simulink model "bmsTestPlatform"  (R2025b)
settings: configuration reference "cfgHarness" (kept outside this file)
PreLoadFcn:
  | if isempty(matlab.project.rootProject)
  |     % Opened outside the project (e.g. by RT-LAB): open it, then return to this folder
  |     d = pwd;
  |     try, openProject(fullfile(d, "..")); catch e, warning(e.message); end
  |     cd(d);
  | end
InitFcn:
  | plant_params
  | sensor_params
  | load_params
undefined symbols (not defined in the file): ADV_tStale, ARB_socTol, batMod, battery_builder_rtmsupport, BMS_state, BMS_stubOut, CAN_Ts, DiscIntNeverNeededParam, f, gcbh, HW_nvm, HW_powerPress, HW_resetPress, HW_rtcStart, LOAD_cycleA, LOAD_cycleAext, LOAD_iConst, LOAD_iPulse, LOAD_profile, LOAD_pulseDuty, LOAD_pulsePeriod, LOAD_scale, PLANT_switchFault, PLANT_tAmbient, PLANT_tContactor, PLANT_Ts, sens, SENS_faultChannel, SENS_faultDuration, SENS_faultRamp, SENS_faultStart, SENS_faultType, SENS_faultValue, SOC0, T0
libraries: bat_13S7P_detailed_lib x7, fl_lib x5, nesl_utility x4, simulink x3, instrumentlib x2
(part 2 of 2)

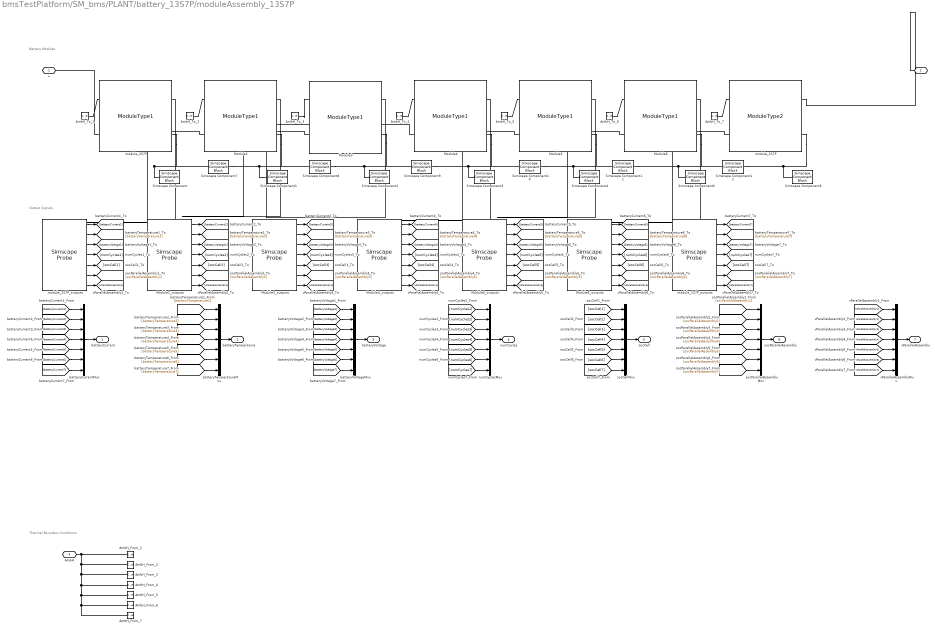
== system bmsTestPlatform/SM_bms/PLANT/battery_13S7P/moduleAssembly_13S7P ==
  note: Thermal Boundary Conditions
  note: Output Signals
  note: Battery Modules
  AmbH_From_1 : ConnectionLabel  Label=ambH_1
  AmbH_From_2 : ConnectionLabel  Label=ambH_2
  AmbH_From_3 : ConnectionLabel  Label=ambH_3
  AmbH_From_4 : ConnectionLabel  Label=ambH_4
  AmbH_From_5 : ConnectionLabel  Label=ambH_5
  AmbH_From_6 : ConnectionLabel  Label=ambH_6
  AmbH_From_7 : ConnectionLabel  Label=ambH_7
  AmbH_To_1 : ConnectionLabel  Label=ambH_1
  AmbH_To_2 : ConnectionLabel  Label=ambH_2
  AmbH_To_3 : ConnectionLabel  Label=ambH_3
  AmbH_To_4 : ConnectionLabel  Label=ambH_4
  AmbH_To_5 : ConnectionLabel  Label=ambH_5
  AmbH_To_6 : ConnectionLabel  Label=ambH_6
  AmbH_To_7 : ConnectionLabel  Label=ambH_7
  Module2 : bat_13S7P_detailed_lib/Modules/ModuleType1  BatteryCapacityCell=batMod(2).BatteryCapacityCell A*hr  ExtrapolationMethodCell=simscape.enum.extrapolation.nearest  SOCBreakpointsCell=batMod(2).SOCBreakpointsCell  TemperatureBreakpointsCell=batMod(2).TemperatureBreakpointsCell K  OpenCircuitVoltageThermalCell=batMod(2).OpenCircuitVoltageThermalCell V  VoltageRangeCell=batMod(2).VoltageRangeCell V  ResistanceSOCBreakpointsCell=batMod(2).ResistanceSOCBreakpointsCell  ResistanceTemperatureBreakpointsCell=batMod(2).ResistanceTemperatureBreakpointsCell K  R0ThermalCell=batMod(2).R0ThermalCell Ohm  R1ThermalCell=batMod(2).R1ThermalCell Ohm  Tau1ThermalCell=batMod(2).Tau1ThermalCell s  BatteryThermalMassCell=batMod(2).BatteryThermalMassCell J/K  AmbientResistance=batMod(2).AmbientResistance K/W  P=7  S=2  socCell_specify=on  socCell_priority=High  socCell=SOC0*ones(14,1)  socCell_nominal_specify=off  socCell_nominal_value=1  socCell_nominal_unit=1  batteryVoltage_specify=off  batteryVoltage_priority=None  batteryVoltage=repmat(0, 14, 1) V  batteryVoltage_nominal_specify=off  batteryVoltage_nominal_value=1  batteryVoltage_nominal_unit=V  batteryCurrent_specify=off  batteryCurrent_priority=None  batteryCurrent=repmat(0, 14, 1) A  batteryCurrent_nominal_specify=off  batteryCurrent_nominal_value=1  batteryCurrent_nominal_unit=A  numCycles_specify=off  numCycles_priority=High  numCycles=repmat(0, 14, 1)  numCycles_nominal_specify=off  numCycles_nominal_value=1  numCycles_nominal_unit=1  batteryTemperature_specify=on  batteryTemperature_priority=High  batteryTemperature=T0*ones(14,1) K  batteryTemperature_nominal_specify=off  batteryTemperature_nominal_value=1  batteryTemperature_nominal_unit=K  vParallelAssembly_specify=off  vParallelAssembly_priority=None  vParallelAssembly=repmat(0, 2, 1) V  vParallelAssembly_nominal_specify=off  vParallelAssembly_nominal_value=1  vParallelAssembly_nominal_unit=V  socParallelAssembly_specify=off  socParallelAssembly_priority=None  socParallelAssembly=repmat(1, 2, 1)  socParallelAssembly_nominal_specify=off  socParallelAssembly_nominal_value=1  socParallelAssembly_nominal_unit=1
      settings: InternalSimscapePortConfiguration="{\"Bottom\":[{\"id\":\"n\",\"label\":\"-\",\"type\":\"foundation.electrical.electrical\"},{\"id\":\"BottomExtClnt\",\"label\":\"CPB\",\"type\":\"foundation.thermal.thermal\"}],\"Left\":[{\"id\":\"AmbH\",\"label\":\"AmbH\",\"type\":\"foundation.thermal.thermal\"}],\"Right\":[],\"Top\":[{\"id\":\"p\",\"label\":\"+\",\"type\":\"foundation.electrical.electrical\"}]}"
  Module2_outputs : SimscapeProbe  BoundBlock=68  Variables="{\"batteryCurrent\":{\"Probing\":\"ON\"},\"batteryTemperature\":{\"Probing\":\"ON\"},\"batteryVoltage\":{\"Probing\":\"ON\"},\"numCycles\":{\"Probing\":\"ON\"},\"socCell\":{\"Probing\":\"ON\"},\"socParallelAssembly\":{\"Probing\":\"ON\"},\"vParallelAssembly\":{\"Probing\":\"ON\"}}"
  Module3 : bat_13S7P_detailed_lib/Modules/ModuleType1  BatteryCapacityCell=batMod(3).BatteryCapacityCell A*hr  ExtrapolationMethodCell=simscape.enum.extrapolation.nearest  SOCBreakpointsCell=batMod(3).SOCBreakpointsCell  TemperatureBreakpointsCell=batMod(3).TemperatureBreakpointsCell K  OpenCircuitVoltageThermalCell=batMod(3).OpenCircuitVoltageThermalCell V  VoltageRangeCell=batMod(3).VoltageRangeCell V  ResistanceSOCBreakpointsCell=batMod(3).ResistanceSOCBreakpointsCell  ResistanceTemperatureBreakpointsCell=batMod(3).ResistanceTemperatureBreakpointsCell K  R0ThermalCell=batMod(3).R0ThermalCell Ohm  R1ThermalCell=batMod(3).R1ThermalCell Ohm  Tau1ThermalCell=batMod(3).Tau1ThermalCell s  BatteryThermalMassCell=batMod(3).BatteryThermalMassCell J/K  AmbientResistance=batMod(3).AmbientResistance K/W  P=7  S=2  socCell_specify=on  socCell_priority=High  socCell=SOC0*ones(14,1)  socCell_nominal_specify=off  socCell_nominal_value=1  socCell_nominal_unit=1  batteryVoltage_specify=off  batteryVoltage_priority=None  batteryVoltage=repmat(0, 14, 1) V  batteryVoltage_nominal_specify=off  batteryVoltage_nominal_value=1  batteryVoltage_nominal_unit=V  batteryCurrent_specify=off  batteryCurrent_priority=None  batteryCurrent=repmat(0, 14, 1) A  batteryCurrent_nominal_specify=off  batteryCurrent_nominal_value=1  batteryCurrent_nominal_unit=A  numCycles_specify=off  numCycles_priority=High  numCycles=repmat(0, 14, 1)  numCycles_nominal_specify=off  numCycles_nominal_value=1  numCycles_nominal_unit=1  batteryTemperature_specify=on  batteryTemperature_priority=High  batteryTemperature=T0*ones(14,1) K  batteryTemperature_nominal_specify=off  batteryTemperature_nominal_value=1  batteryTemperature_nominal_unit=K  vParallelAssembly_specify=off  vParallelAssembly_priority=None  vParallelAssembly=repmat(0, 2, 1) V  vParallelAssembly_nominal_specify=off  vParallelAssembly_nominal_value=1  vParallelAssembly_nominal_unit=V  socParallelAssembly_specify=off  socParallelAssembly_priority=None  socParallelAssembly=repmat(1, 2, 1)  socParallelAssembly_nominal_specify=off  socParallelAssembly_nominal_value=1  socParallelAssembly_nominal_unit=1
      settings: InternalSimscapePortConfiguration="{\"Bottom\":[{\"id\":\"n\",\"label\":\"-\",\"type\":\"foundation.electrical.electrical\"},{\"id\":\"BottomExtClnt\",\"label\":\"CPB\",\"type\":\"foundation.thermal.thermal\"}],\"Left\":[{\"id\":\"AmbH\",\"label\":\"AmbH\",\"type\":\"foundation.thermal.thermal\"}],\"Right\":[],\"Top\":[{\"id\":\"p\",\"label\":\"+\",\"type\":\"foundation.electrical.electrical\"}]}"
  Module3_outputs : SimscapeProbe  BoundBlock=70  Variables="{\"batteryCurrent\":{\"Probing\":\"ON\"},\"batteryTemperature\":{\"Probing\":\"ON\"},\"batteryVoltage\":{\"Probing\":\"ON\"},\"numCycles\":{\"Probing\":\"ON\"},\"socCell\":{\"Probing\":\"ON\"},\"socParallelAssembly\":{\"Probing\":\"ON\"},\"vParallelAssembly\":{\"Probing\":\"ON\"}}"
  Module4 : bat_13S7P_detailed_lib/Modules/ModuleType1  BatteryCapacityCell=batMod(4).BatteryCapacityCell A*hr  ExtrapolationMethodCell=simscape.enum.extrapolation.nearest  SOCBreakpointsCell=batMod(4).SOCBreakpointsCell  TemperatureBreakpointsCell=batMod(4).TemperatureBreakpointsCell K  OpenCircuitVoltageThermalCell=batMod(4).OpenCircuitVoltageThermalCell V  VoltageRangeCell=batMod(4).VoltageRangeCell V  ResistanceSOCBreakpointsCell=batMod(4).ResistanceSOCBreakpointsCell  ResistanceTemperatureBreakpointsCell=batMod(4).ResistanceTemperatureBreakpointsCell K  R0ThermalCell=batMod(4).R0ThermalCell Ohm  R1ThermalCell=batMod(4).R1ThermalCell Ohm  Tau1ThermalCell=batMod(4).Tau1ThermalCell s  BatteryThermalMassCell=batMod(4).BatteryThermalMassCell J/K  AmbientResistance=batMod(4).AmbientResistance K/W  P=7  S=2  socCell_specify=on  socCell_priority=High  socCell=SOC0*ones(14,1)  socCell_nominal_specify=off  socCell_nominal_value=1  socCell_nominal_unit=1  batteryVoltage_specify=off  batteryVoltage_priority=None  batteryVoltage=repmat(0, 14, 1) V  batteryVoltage_nominal_specify=off  batteryVoltage_nominal_value=1  batteryVoltage_nominal_unit=V  batteryCurrent_specify=off  batteryCurrent_priority=None  batteryCurrent=repmat(0, 14, 1) A  batteryCurrent_nominal_specify=off  batteryCurrent_nominal_value=1  batteryCurrent_nominal_unit=A  numCycles_specify=off  numCycles_priority=High  numCycles=repmat(0, 14, 1)  numCycles_nominal_specify=off  numCycles_nominal_value=1  numCycles_nominal_unit=1  batteryTemperature_specify=on  batteryTemperature_priority=High  batteryTemperature=T0*ones(14,1) K  batteryTemperature_nominal_specify=off  batteryTemperature_nominal_value=1  batteryTemperature_nominal_unit=K  vParallelAssembly_specify=off  vParallelAssembly_priority=None  vParallelAssembly=repmat(0, 2, 1) V  vParallelAssembly_nominal_specify=off  vParallelAssembly_nominal_value=1  vParallelAssembly_nominal_unit=V  socParallelAssembly_specify=off  socParallelAssembly_priority=None  socParallelAssembly=repmat(1, 2, 1)  socParallelAssembly_nominal_specify=off  socParallelAssembly_nominal_value=1  socParallelAssembly_nominal_unit=1
      settings: InternalSimscapePortConfiguration="{\"Bottom\":[{\"id\":\"n\",\"label\":\"-\",\"type\":\"foundation.electrical.electrical\"},{\"id\":\"BottomExtClnt\",\"label\":\"CPB\",\"type\":\"foundation.thermal.thermal\"}],\"Left\":[{\"id\":\"AmbH\",\"label\":\"AmbH\",\"type\":\"foundation.thermal.thermal\"}],\"Right\":[],\"Top\":[{\"id\":\"p\",\"label\":\"+\",\"type\":\"foundation.electrical.electrical\"}]}"
  Module4_outputs : SimscapeProbe  BoundBlock=72  Variables="{\"batteryCurrent\":{\"Probing\":\"ON\"},\"batteryTemperature\":{\"Probing\":\"ON\"},\"batteryVoltage\":{\"Probing\":\"ON\"},\"numCycles\":{\"Probing\":\"ON\"},\"socCell\":{\"Probing\":\"ON\"},\"socParallelAssembly\":{\"Probing\":\"ON\"},\"vParallelAssembly\":{\"Probing\":\"ON\"}}"
  Module5 : bat_13S7P_detailed_lib/Modules/ModuleType1  BatteryCapacityCell=batMod(5).BatteryCapacityCell A*hr  ExtrapolationMethodCell=simscape.enum.extrapolation.nearest  SOCBreakpointsCell=batMod(5).SOCBreakpointsCell  TemperatureBreakpointsCell=batMod(5).TemperatureBreakpointsCell K  OpenCircuitVoltageThermalCell=batMod(5).OpenCircuitVoltageThermalCell V  VoltageRangeCell=batMod(5).VoltageRangeCell V  ResistanceSOCBreakpointsCell=batMod(5).ResistanceSOCBreakpointsCell  ResistanceTemperatureBreakpointsCell=batMod(5).ResistanceTemperatureBreakpointsCell K  R0ThermalCell=batMod(5).R0ThermalCell Ohm  R1ThermalCell=batMod(5).R1ThermalCell Ohm  Tau1ThermalCell=batMod(5).Tau1ThermalCell s  BatteryThermalMassCell=batMod(5).BatteryThermalMassCell J/K  AmbientResistance=batMod(5).AmbientResistance K/W  P=7  S=2  socCell_specify=on  socCell_priority=High  socCell=SOC0*ones(14,1)  socCell_nominal_specify=off  socCell_nominal_value=1  socCell_nominal_unit=1  batteryVoltage_specify=off  batteryVoltage_priority=None  batteryVoltage=repmat(0, 14, 1) V  batteryVoltage_nominal_specify=off  batteryVoltage_nominal_value=1  batteryVoltage_nominal_unit=V  batteryCurrent_specify=off  batteryCurrent_priority=None  batteryCurrent=repmat(0, 14, 1) A  batteryCurrent_nominal_specify=off  batteryCurrent_nominal_value=1  batteryCurrent_nominal_unit=A  numCycles_specify=off  numCycles_priority=High  numCycles=repmat(0, 14, 1)  numCycles_nominal_specify=off  numCycles_nominal_value=1  numCycles_nominal_unit=1  batteryTemperature_specify=on  batteryTemperature_priority=High  batteryTemperature=T0*ones(14,1) K  batteryTemperature_nominal_specify=off  batteryTemperature_nominal_value=1  batteryTemperature_nominal_unit=K  vParallelAssembly_specify=off  vParallelAssembly_priority=None  vParallelAssembly=repmat(0, 2, 1) V  vParallelAssembly_nominal_specify=off  vParallelAssembly_nominal_value=1  vParallelAssembly_nominal_unit=V  socParallelAssembly_specify=off  socParallelAssembly_priority=None  socParallelAssembly=repmat(1, 2, 1)  socParallelAssembly_nominal_specify=off  socParallelAssembly_nominal_value=1  socParallelAssembly_nominal_unit=1
      settings: InternalSimscapePortConfiguration="{\"Bottom\":[{\"id\":\"n\",\"label\":\"-\",\"type\":\"foundation.electrical.electrical\"},{\"id\":\"BottomExtClnt\",\"label\":\"CPB\",\"type\":\"foundation.thermal.thermal\"}],\"Left\":[{\"id\":\"AmbH\",\"label\":\"AmbH\",\"type\":\"foundation.thermal.thermal\"}],\"Right\":[],\"Top\":[{\"id\":\"p\",\"label\":\"+\",\"type\":\"foundation.electrical.electrical\"}]}"
  Module5_outputs : SimscapeProbe  BoundBlock=74  Variables="{\"batteryCurrent\":{\"Probing\":\"ON\"},\"batteryTemperature\":{\"Probing\":\"ON\"},\"batteryVoltage\":{\"Probing\":\"ON\"},\"numCycles\":{\"Probing\":\"ON\"},\"socCell\":{\"Probing\":\"ON\"},\"socParallelAssembly\":{\"Probing\":\"ON\"},\"vParallelAssembly\":{\"Probing\":\"ON\"}}"
  Module6 : bat_13S7P_detailed_lib/Modules/ModuleType1  BatteryCapacityCell=batMod(6).BatteryCapacityCell A*hr  ExtrapolationMethodCell=simscape.enum.extrapolation.nearest  SOCBreakpointsCell=batMod(6).SOCBreakpointsCell  TemperatureBreakpointsCell=batMod(6).TemperatureBreakpointsCell K  OpenCircuitVoltageThermalCell=batMod(6).OpenCircuitVoltageThermalCell V  VoltageRangeCell=batMod(6).VoltageRangeCell V  ResistanceSOCBreakpointsCell=batMod(6).ResistanceSOCBreakpointsCell  ResistanceTemperatureBreakpointsCell=batMod(6).ResistanceTemperatureBreakpointsCell K  R0ThermalCell=batMod(6).R0ThermalCell Ohm  R1ThermalCell=batMod(6).R1ThermalCell Ohm  Tau1ThermalCell=batMod(6).Tau1ThermalCell s  BatteryThermalMassCell=batMod(6).BatteryThermalMassCell J/K  AmbientResistance=batMod(6).AmbientResistance K/W  P=7  S=2  socCell_specify=on  socCell_priority=High  socCell=SOC0*ones(14,1)  socCell_nominal_specify=off  socCell_nominal_value=1  socCell_nominal_unit=1  batteryVoltage_specify=off  batteryVoltage_priority=None  batteryVoltage=repmat(0, 14, 1) V  batteryVoltage_nominal_specify=off  batteryVoltage_nominal_value=1  batteryVoltage_nominal_unit=V  batteryCurrent_specify=off  batteryCurrent_priority=None  batteryCurrent=repmat(0, 14, 1) A  batteryCurrent_nominal_specify=off  batteryCurrent_nominal_value=1  batteryCurrent_nominal_unit=A  numCycles_specify=off  numCycles_priority=High  numCycles=repmat(0, 14, 1)  numCycles_nominal_specify=off  numCycles_nominal_value=1  numCycles_nominal_unit=1  batteryTemperature_specify=on  batteryTemperature_priority=High  batteryTemperature=T0*ones(14,1) K  batteryTemperature_nominal_specify=off  batteryTemperature_nominal_value=1  batteryTemperature_nominal_unit=K  vParallelAssembly_specify=off  vParallelAssembly_priority=None  vParallelAssembly=repmat(0, 2, 1) V  vParallelAssembly_nominal_specify=off  vParallelAssembly_nominal_value=1  vParallelAssembly_nominal_unit=V  socParallelAssembly_specify=off  socParallelAssembly_priority=None  socParallelAssembly=repmat(1, 2, 1)  socParallelAssembly_nominal_specify=off  socParallelAssembly_nominal_value=1  socParallelAssembly_nominal_unit=1
      settings: InternalSimscapePortConfiguration="{\"Bottom\":[{\"id\":\"n\",\"label\":\"-\",\"type\":\"foundation.electrical.electrical\"},{\"id\":\"BottomExtClnt\",\"label\":\"CPB\",\"type\":\"foundation.thermal.thermal\"}],\"Left\":[{\"id\":\"AmbH\",\"label\":\"AmbH\",\"type\":\"foundation.thermal.thermal\"}],\"Right\":[],\"Top\":[{\"id\":\"p\",\"label\":\"+\",\"type\":\"foundation.electrical.electrical\"}]}"
  Module6_outputs : SimscapeProbe  BoundBlock=76  Variables="{\"batteryCurrent\":{\"Probing\":\"ON\"},\"batteryTemperature\":{\"Probing\":\"ON\"},\"batteryVoltage\":{\"Probing\":\"ON\"},\"numCycles\":{\"Probing\":\"ON\"},\"socCell\":{\"Probing\":\"ON\"},\"socParallelAssembly\":{\"Probing\":\"ON\"},\"vParallelAssembly\":{\"Probing\":\"ON\"}}"
  Simscape Component{,1..5} (6 alike) : SimscapeComponentBlock  SourceFile=cellPairs_2S7P  ComponentPath=cellPairs_2S7P  ComponentVariants="[\"cellPairs_2S7P\"]"  ComponentVariantNames="[\"cellPairs_2S7P\"]"  ClassName=cellPairs_2S7P  SchemaVersion=1  R=[61.73, 54.15, 61.73, 57.32, 61.72, 58.62, 58.63, 55.64, 58.64, 55.64, 58.63, 61.72, 58.62, 57.32, 54.15, 61.73, 61.73] K/W
      settings: CopyFcn=simscape.sscblock.internal.componentBlockCallback(gcbh,'COPY')  PreCopyFcn=simscape.sscblock.internal.componentBlockCallback(gcbh,'PRECOPY')  PreDeleteFcn=simscape.sscblock.internal.componentBlockCallback(gcbh,'PREDELETE')  InternalSimscapePortConfiguration="{\"Bottom\":[],\"Left\":[{\"id\":\"H\",\"label\":\"H\",\"type\":\"foundation.thermal.thermal\"}],\"Right\":[],\"Top\":[]}"
      mask Type: Cell-to-cell thermal network within one 2S7P slice (14 cells, 17 neighbour pairs).
  Simscape Component{7..11} (5 alike) : SimscapeComponentBlock  SourceFile=axialLink_2S7P  ComponentPath=axialLink_2S7P  ComponentVariants="[\"axialLink_2S7P\"]"  ComponentVariantNames="[\"axialLink_2S7P\"]"  ClassName=axialLink_2S7P  SchemaVersion=1  R=180.4 K/W
      settings: CopyFcn=simscape.sscblock.internal.componentBlockCallback(gcbh,'COPY')  PreCopyFcn=simscape.sscblock.internal.componentBlockCallback(gcbh,'PRECOPY')  PreDeleteFcn=simscape.sscblock.internal.componentBlockCallback(gcbh,'PREDELETE')  InternalSimscapePortConfiguration="{\"Bottom\":[],\"Left\":[{\"id\":\"A\",\"label\":\"A\",\"type\":\"foundation.thermal.thermal\"}],\"Right\":[{\"id\":\"B\",\"label\":\"B\",\"type\":\"foundation.thermal.thermal\"}],\"Top\":[]}"
      mask Type: Slice-to-slice thermal links
  Simscape Component12 : SimscapeComponentBlock  SourceFile=axialLink_2S7P_1S7P  ComponentPath=axialLink_2S7P_1S7P  ComponentVariants="[\"axialLink_2S7P_1S7P\"]"  ComponentVariantNames="[\"axialLink_2S7P_1S7P\"]"  ClassName=axialLink_2S7P_1S7P  SchemaVersion=1  R=180.4 K/W
      settings: CopyFcn=simscape.sscblock.internal.componentBlockCallback(gcbh,'COPY')  PreCopyFcn=simscape.sscblock.internal.componentBlockCallback(gcbh,'PRECOPY')  PreDeleteFcn=simscape.sscblock.internal.componentBlockCallback(gcbh,'PREDELETE')  InternalSimscapePortConfiguration="{\"Bottom\":[],\"Left\":[{\"id\":\"A\",\"label\":\"A\",\"type\":\"foundation.thermal.thermal\"}],\"Right\":[{\"id\":\"B\",\"label\":\"B\",\"type\":\"foundation.thermal.thermal\"}],\"Top\":[]}"
      mask Type: Slice-to-slice thermal links
  Simscape Component6 : SimscapeComponentBlock  SourceFile=cellPairs_1S7P  ComponentPath=cellPairs_1S7P  ComponentVariants="[\"cellPairs_1S7P\"]"  ComponentVariantNames="[\"cellPairs_1S7P\"]"  ClassName=cellPairs_1S7P  SchemaVersion=1  R=[61.73, 54.15, 61.73, 57.32, 61.72, 58.62, 58.63, 55.64] K/W
      settings: CopyFcn=simscape.sscblock.internal.componentBlockCallback(gcbh,'COPY')  PreCopyFcn=simscape.sscblock.internal.componentBlockCallback(gcbh,'PRECOPY')  PreDeleteFcn=simscape.sscblock.internal.componentBlockCallback(gcbh,'PREDELETE')  InternalSimscapePortConfiguration="{\"Bottom\":[],\"Left\":[{\"id\":\"H\",\"label\":\"H\",\"type\":\"foundation.thermal.thermal\"}],\"Right\":[],\"Top\":[]}"
      mask Type: Cell-to-cell thermal network within one 1S7P slice (7 cells, 8 neighbour pairs).
  batteryCurrentMux : Mux  Inputs=7
  batteryTemperatureMux : Mux  Inputs=7
  batteryVoltageMux : Mux  Inputs=7
  module_1S7P : bat_13S7P_detailed_lib/Modules/ModuleType2  BatteryCapacityCell=batMod(7).BatteryCapacityCell A*hr  ExtrapolationMethodCell=simscape.enum.extrapolation.nearest  SOCBreakpointsCell=batMod(7).SOCBreakpointsCell  TemperatureBreakpointsCell=batMod(7).TemperatureBreakpointsCell K  OpenCircuitVoltageThermalCell=batMod(7).OpenCircuitVoltageThermalCell V  VoltageRangeCell=batMod(7).VoltageRangeCell V  ResistanceSOCBreakpointsCell=batMod(7).ResistanceSOCBreakpointsCell  ResistanceTemperatureBreakpointsCell=batMod(7).ResistanceTemperatureBreakpointsCell K  R0ThermalCell=batMod(7).R0ThermalCell Ohm  R1ThermalCell=batMod(7).R1ThermalCell Ohm  Tau1ThermalCell=batMod(7).Tau1ThermalCell s  BatteryThermalMassCell=batMod(7).BatteryThermalMassCell J/K  AmbientResistance=batMod(7).AmbientResistance K/W  P=7  S=1  socCell_specify=on  socCell_priority=High  socCell=SOC0*ones(7,1)  socCell_nominal_specify=off  socCell_nominal_value=1  socCell_nominal_unit=1  batteryVoltage_specify=off  batteryVoltage_priority=None  batteryVoltage=repmat(0, 7, 1) V  batteryVoltage_nominal_specify=off  batteryVoltage_nominal_value=1  batteryVoltage_nominal_unit=V  batteryCurrent_specify=off  batteryCurrent_priority=None  batteryCurrent=repmat(0, 7, 1) A  batteryCurrent_nominal_specify=off  batteryCurrent_nominal_value=1  batteryCurrent_nominal_unit=A  numCycles_specify=off  numCycles_priority=High  numCycles=repmat(0, 7, 1)  numCycles_nominal_specify=off  numCycles_nominal_value=1  numCycles_nominal_unit=1  batteryTemperature_specify=on  batteryTemperature_priority=High  batteryTemperature=T0*ones(7,1) K  batteryTemperature_nominal_specify=off  batteryTemperature_nominal_value=1  batteryTemperature_nominal_unit=K  vParallelAssembly_specify=off  vParallelAssembly_priority=None  vParallelAssembly=0 V  vParallelAssembly_nominal_specify=off  vParallelAssembly_nominal_value=1  vParallelAssembly_nominal_unit=V  socParallelAssembly_specify=off  socParallelAssembly_priority=None  socParallelAssembly=1  socParallelAssembly_nominal_specify=off  socParallelAssembly_nominal_value=1  socParallelAssembly_nominal_unit=1
      settings: InternalSimscapePortConfiguration="{\"Bottom\":[{\"id\":\"n\",\"label\":\"-\",\"type\":\"foundation.electrical.electrical\"},{\"id\":\"BottomExtClnt\",\"label\":\"CPB\",\"type\":\"foundation.thermal.thermal\"}],\"Left\":[{\"id\":\"AmbH\",\"label\":\"AmbH\",\"type\":\"foundation.thermal.thermal\"}],\"Right\":[],\"Top\":[{\"id\":\"p\",\"label\":\"+\",\"type\":\"foundation.electrical.electrical\"}]}"
  module_1S7P_outputs : SimscapeProbe  BoundBlock=123  Variables="{\"batteryCurrent\":{\"Probing\":\"ON\"},\"batteryTemperature\":{\"Probing\":\"ON\"},\"batteryVoltage\":{\"Probing\":\"ON\"},\"numCycles\":{\"Probing\":\"ON\"},\"socCell\":{\"Probing\":\"ON\"},\"socParallelAssembly\":{\"Probing\":\"ON\"},\"vParallelAssembly\":{\"Probing\":\"ON\"}}"
  module_2S7P : bat_13S7P_detailed_lib/Modules/ModuleType1  BatteryCapacityCell=batMod(1).BatteryCapacityCell A*hr  ExtrapolationMethodCell=simscape.enum.extrapolation.nearest  SOCBreakpointsCell=batMod(1).SOCBreakpointsCell  TemperatureBreakpointsCell=batMod(1).TemperatureBreakpointsCell K  OpenCircuitVoltageThermalCell=batMod(1).OpenCircuitVoltageThermalCell V  VoltageRangeCell=batMod(1).VoltageRangeCell V  ResistanceSOCBreakpointsCell=batMod(1).ResistanceSOCBreakpointsCell  ResistanceTemperatureBreakpointsCell=batMod(1).ResistanceTemperatureBreakpointsCell K  R0ThermalCell=batMod(1).R0ThermalCell Ohm  R1ThermalCell=batMod(1).R1ThermalCell Ohm  Tau1ThermalCell=batMod(1).Tau1ThermalCell s  BatteryThermalMassCell=batMod(1).BatteryThermalMassCell J/K  AmbientResistance=batMod(1).AmbientResistance K/W  P=7  S=2  socCell_specify=on  socCell_priority=High  socCell=SOC0*ones(14,1)  socCell_nominal_specify=off  socCell_nominal_value=1  socCell_nominal_unit=1  batteryVoltage_specify=off  batteryVoltage_priority=None  batteryVoltage=repmat(0, 14, 1) V  batteryVoltage_nominal_specify=off  batteryVoltage_nominal_value=1  batteryVoltage_nominal_unit=V  batteryCurrent_specify=off  batteryCurrent_priority=None  batteryCurrent=repmat(0, 14, 1) A  batteryCurrent_nominal_specify=off  batteryCurrent_nominal_value=1  batteryCurrent_nominal_unit=A  numCycles_specify=off  numCycles_priority=High  numCycles=repmat(0, 14, 1)  numCycles_nominal_specify=off  numCycles_nominal_value=1  numCycles_nominal_unit=1  batteryTemperature_specify=on  batteryTemperature_priority=High  batteryTemperature=T0*ones(14,1) K  batteryTemperature_nominal_specify=off  batteryTemperature_nominal_value=1  batteryTemperature_nominal_unit=K  vParallelAssembly_specify=off  vParallelAssembly_priority=None  vParallelAssembly=repmat(0, 2, 1) V  vParallelAssembly_nominal_specify=off  vParallelAssembly_nominal_value=1  vParallelAssembly_nominal_unit=V  socParallelAssembly_specify=off  socParallelAssembly_priority=None  socParallelAssembly=repmat(1, 2, 1)  socParallelAssembly_nominal_specify=off  socParallelAssembly_nominal_value=1  socParallelAssembly_nominal_unit=1
      settings: InternalSimscapePortConfiguration="{\"Bottom\":[{\"id\":\"n\",\"label\":\"-\",\"type\":\"foundation.electrical.electrical\"},{\"id\":\"BottomExtClnt\",\"label\":\"CPB\",\"type\":\"foundation.thermal.thermal\"}],\"Left\":[{\"id\":\"AmbH\",\"label\":\"AmbH\",\"type\":\"foundation.thermal.thermal\"}],\"Right\":[],\"Top\":[{\"id\":\"p\",\"label\":\"+\",\"type\":\"foundation.electrical.electrical\"}]}"
  module_2S7P_outputs : SimscapeProbe  BoundBlock=125  Variables="{\"batteryCurrent\":{\"Probing\":\"ON\"},\"batteryTemperature\":{\"Probing\":\"ON\"},\"batteryVoltage\":{\"Probing\":\"ON\"},\"numCycles\":{\"Probing\":\"ON\"},\"socCell\":{\"Probing\":\"ON\"},\"socParallelAssembly\":{\"Probing\":\"ON\"},\"vParallelAssembly\":{\"Probing\":\"ON\"}}"
  numCyclesMux : Mux  Inputs=7
  socCellMux : Mux  Inputs=7
  socParallelAssemblyMux : Mux  Inputs=7
  vParallelAssemblyMux : Mux  Inputs=7
  + : PMIOPort  Side=Left
  - : PMIOPort  Port=2  Side=Right
  AmbH : PMIOPort  Port=3  Side=Right  ConnectionType=Connection: foundation.thermal.thermal
  batteryCurrent : Outport
  batteryTemperature : Outport  Port=2
  batteryVoltage : Outport  Port=3
  numCycles : Outport  Port=4
  socCell : Outport  Port=5
  socParallelAssembly : Outport  Port=6
  vParallelAssembly : Outport  Port=7
  wires:
  [vParallelAssembly7] -> vParallelAssemblyMux/7
  module_1S7P_outputs/7 -> [vParallelAssembly7]
  [socParallelAssembly7] -> socParallelAssemblyMux/7
  module_1S7P_outputs/6 -> [socParallelAssembly7]
  [socCell7] -> socCellMux/7
  module_1S7P_outputs/5 -> [socCell7]
  [numCycles7] -> numCyclesMux/7
  module_1S7P_outputs/4 -> [numCycles7]
  [batteryVoltage7] -> batteryVoltageMux/7
  module_1S7P_outputs/3 -> [batteryVoltage7]
  [batteryTemperature7] -> batteryTemperatureMux/7
  module_1S7P_outputs/2 -> [batteryTemperature7]
  [batteryCurrent7] -> batteryCurrentMux/7
  module_1S7P_outputs/1 -> [batteryCurrent7]
  [vParallelAssembly6] -> vParallelAssemblyMux/6
  Module6_outputs/7 -> [vParallelAssembly6]
  [socParallelAssembly6] -> socParallelAssemblyMux/6
  Module6_outputs/6 -> [socParallelAssembly6]
  [socCell6] -> socCellMux/6
  Module6_outputs/5 -> [socCell6]
  [numCycles6] -> numCyclesMux/6
  Module6_outputs/4 -> [numCycles6]
  [batteryVoltage6] -> batteryVoltageMux/6
  Module6_outputs/3 -> [batteryVoltage6]
  [batteryTemperature6] -> batteryTemperatureMux/6
  Module6_outputs/2 -> [batteryTemperature6]
  [batteryCurrent6] -> batteryCurrentMux/6
  Module6_outputs/1 -> [batteryCurrent6]
  [vParallelAssembly5] -> vParallelAssemblyMux/5
  Module5_outputs/7 -> [vParallelAssembly5]
  [socParallelAssembly5] -> socParallelAssemblyMux/5
  Module5_outputs/6 -> [socParallelAssembly5]
  [socCell5] -> socCellMux/5
  Module5_outputs/5 -> [socCell5]
  [numCycles5] -> numCyclesMux/5
  Module5_outputs/4 -> [numCycles5]
  [batteryVoltage5] -> batteryVoltageMux/5
  Module5_outputs/3 -> [batteryVoltage5]
  [batteryTemperature5] -> batteryTemperatureMux/5
  Module5_outputs/2 -> [batteryTemperature5]
  [batteryCurrent5] -> batteryCurrentMux/5
  Module5_outputs/1 -> [batteryCurrent5]
  [vParallelAssembly4] -> vParallelAssemblyMux/4
  Module4_outputs/7 -> [vParallelAssembly4]
  [socParallelAssembly4] -> socParallelAssemblyMux/4
  Module4_outputs/6 -> [socParallelAssembly4]
  [socCell4] -> socCellMux/4
  Module4_outputs/5 -> [socCell4]
  [numCycles4] -> numCyclesMux/4
  Module4_outputs/4 -> [numCycles4]
  [batteryVoltage4] -> batteryVoltageMux/4
  Module4_outputs/3 -> [batteryVoltage4]
  [batteryTemperature4] -> batteryTemperatureMux/4
  Module4_outputs/2 -> [batteryTemperature4]
  [batteryCurrent4] -> batteryCurrentMux/4
  Module4_outputs/1 -> [batteryCurrent4]
  [vParallelAssembly3] -> vParallelAssemblyMux/3
  Module3_outputs/7 -> [vParallelAssembly3]
  [socParallelAssembly3] -> socParallelAssemblyMux/3
  Module3_outputs/6 -> [socParallelAssembly3]
  [socCell3] -> socCellMux/3
  Module3_outputs/5 -> [socCell3]
  [numCycles3] -> numCyclesMux/3
  Module3_outputs/4 -> [numCycles3]
  [batteryVoltage3] -> batteryVoltageMux/3
  Module3_outputs/3 -> [batteryVoltage3]
  [batteryTemperature3] -> batteryTemperatureMux/3
  Module3_outputs/2 -> [batteryTemperature3]
  [batteryCurrent3] -> batteryCurrentMux/3
  Module3_outputs/1 -> [batteryCurrent3]
  [vParallelAssembly2] -> vParallelAssemblyMux/2
  Module2_outputs/7 -> [vParallelAssembly2]
  [socParallelAssembly2] -> socParallelAssemblyMux/2
  Module2_outputs/6 -> [socParallelAssembly2]
  [socCell2] -> socCellMux/2
  Module2_outputs/5 -> [socCell2]
  [numCycles2] -> numCyclesMux/2
  Module2_outputs/4 -> [numCycles2]
  [batteryVoltage2] -> batteryVoltageMux/2
  Module2_outputs/3 -> [batteryVoltage2]
  [batteryTemperature2] -> batteryTemperatureMux/2
  Module2_outputs/2 -> [batteryTemperature2]
  [batteryCurrent2] -> batteryCurrentMux/2
  Module2_outputs/1 -> [batteryCurrent2]
  [vParallelAssembly1] -> vParallelAssemblyMux/1
  vParallelAssemblyMux/1 -> vParallelAssembly/1
  module_2S7P_outputs/7 -> [vParallelAssembly1]
  [socParallelAssembly1] -> socParallelAssemblyMux/1
  socParallelAssemblyMux/1 -> socParallelAssembly/1
  module_2S7P_outputs/6 -> [socParallelAssembly1]
  [socCell1] -> socCellMux/1
  socCellMux/1 -> socCell/1
  module_2S7P_outputs/5 -> [socCell1]
  [numCycles1] -> numCyclesMux/1
  numCyclesMux/1 -> numCycles/1
  module_2S7P_outputs/4 -> [numCycles1]
  [batteryVoltage1] -> batteryVoltageMux/1
  batteryVoltageMux/1 -> batteryVoltage/1
  module_2S7P_outputs/3 -> [batteryVoltage1]
  [batteryTemperature1] -> batteryTemperatureMux/1
  batteryTemperatureMux/1 -> batteryTemperature/1
  module_2S7P_outputs/2 -> [batteryTemperature1]
  [batteryCurrent1] -> batteryCurrentMux/1
  batteryCurrentMux/1 -> batteryCurrent/1
  module_2S7P_outputs/1 -> [batteryCurrent1]
  connections:
  AmbH_To_7/LConn1 -- module_1S7P/LConn1
  AmbH_To_6/LConn1 -- Module6/LConn1
  AmbH_To_5/LConn1 -- Module5/LConn1
  AmbH_To_4/LConn1 -- Module4/LConn1
  AmbH_To_3/LConn1 -- Module3/LConn1
  AmbH_To_2/LConn1 -- Module2/LConn1
  AmbH_From_7/LConn1 -- AmbH/RConn1 -- AmbH_From_1/LConn1 -- AmbH_From_2/LConn1 -- AmbH_From_3/LConn1 -- AmbH_From_4/LConn1 -- AmbH_From_5/LConn1 -- AmbH_From_6/LConn1
  AmbH_To_1/LConn1 -- module_2S7P/LConn1
  module_1S7P/RConn1 -- -/RConn1
  module_2S7P/LConn2 -- +/RConn1
  module_1S7P/LConn2 -- Module6/RConn1
  Module6/LConn2 -- Module5/RConn1
  Module5/LConn2 -- Module4/RConn1
  Module4/LConn2 -- Module3/RConn1
  Module3/LConn2 -- Module2/RConn1
  Module2/LConn2 -- module_2S7P/RConn1
  Simscape Component10/RConn1 -- Module5/RConn2 -- Simscape Component4/LConn1 -- Simscape Component11/LConn1
  Simscape Component/LConn1 -- module_2S7P/RConn2 -- Simscape Component7/LConn1
  Simscape Component1/LConn1 -- Module2/RConn2 -- Simscape Component8/LConn1 -- Simscape Component7/RConn1
  Simscape Component9/RConn1 -- Module4/RConn2 -- Simscape Component3/LConn1 -- Simscape Component10/LConn1
  Simscape Component2/LConn1 -- Module3/RConn2 -- Simscape Component9/LConn1 -- Simscape Component8/RConn1
  Simscape Component12/RConn1 -- module_1S7P/RConn2 -- Simscape Component6/LConn1
  Simscape Component11/RConn1 -- Module6/RConn2 -- Simscape Component5/LConn1 -- Simscape Component12/LConn1

== matlab function bmsTestPlatform/SM_bms/BMS_HW/hwFcn ==
  data: t input double; hw output Bus: BMS_hwIn; bmsState input Enum: BMS_state; nvmSaved input Bus: BMS_nvmRecord; HW_rtcStart parameter; HW_nvm parameter; HW_powerPress parameter; HW_resetPress parameter
function hw = hwFcn(t, bmsState, nvmSaved, HW_rtcStart, HW_nvm, HW_powerPress, HW_resetPress)
% Platform stand-in for the BMS board peripherals: clock, non-volatile memory, buttons. Logic in hwEmulator.m.
hw = hwEmulator(t, bmsState, nvmSaved, HW_rtcStart, HW_nvm, HW_powerPress, HW_resetPress);

== matlab function bmsTestPlatform/SM_bms/SENS_FAULT/faultFcn ==
  data: m input Bus: SENS_measBus; mOut output Bus: SENS_measBus; SENS_faultType parameter; SENS_faultChannel parameter; SENS_faultValue parameter; SENS_faultStart parameter; SENS_faultDuration parameter; SENS_faultRamp parameter
function mOut = faultFcn(m, SENS_faultType, SENS_faultChannel, SENS_faultValue, SENS_faultStart, SENS_faultDuration, SENS_faultRamp)
% Platform-only measurement fault injection. Logic in sensFaultInject.m.
mOut = sensFaultInject(m, SENS_faultType, SENS_faultChannel, SENS_faultValue, SENS_faultStart, SENS_faultDuration, SENS_faultRamp);

== matlab function bmsTestPlatform/SM_bms/CAN/NONE/advStub ==
  data: adv output Bus: ADV_bus; CAN_Ts parameter; ADV_tStale parameter
function adv = advNone(CAN_Ts, ADV_tStale)
% no estimator connected: canRx with no data (not fresh, not valid, NaN values)
adv = canRx(zeros(128, 1, 'uint8'), false, CAN_Ts, ADV_tStale);

== matlab function bmsTestPlatform/SM_bms/CAN/UDP/canTx ==
  data: b input Bus: BMS_outBus; frames output uint8 size=[208 1]; CAN_bmsLim parameter
function frames = canTxBlk(b, CAN_bmsLim)
% BMS outputs -> 13 CAN frames (Linux can_frame records) for UDP; see canTx.m
frames = canTx(b, CAN_bmsLim);

== matlab function bmsTestPlatform/SM_bms/CAN/UDP/canRx ==
  data: data input uint8 size=[128 1]; adv output Bus: ADV_bus; status input; CAN_Ts parameter; ADV_tStale parameter
function adv = canRxBlk(data, status, CAN_Ts, ADV_tStale)
% advisory frames from the Pi -> ADV_bus; see canRx.m
adv = canRx(data, status > 0, CAN_Ts, ADV_tStale);
